simulink model "activeControlSimcopycopy"  (R2026a)
settings: Solver=ode4  StopTime=35  FixedStep=0.01
settings Model: DataDictionary=navParams.sldd  PauseTimes=2  Creator=maxhu  LastModifiedBy=nathanscott

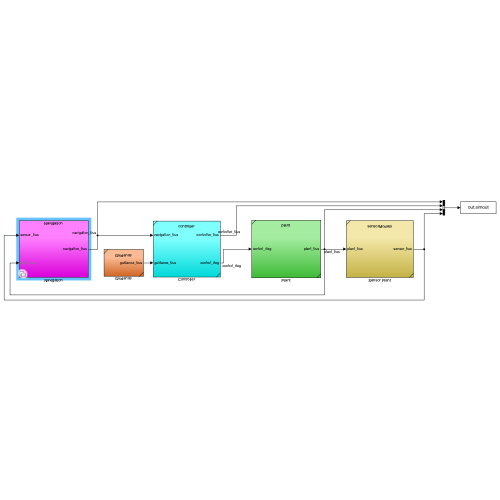
[thumbnail: Simulink's stored preview of the top-level diagram]
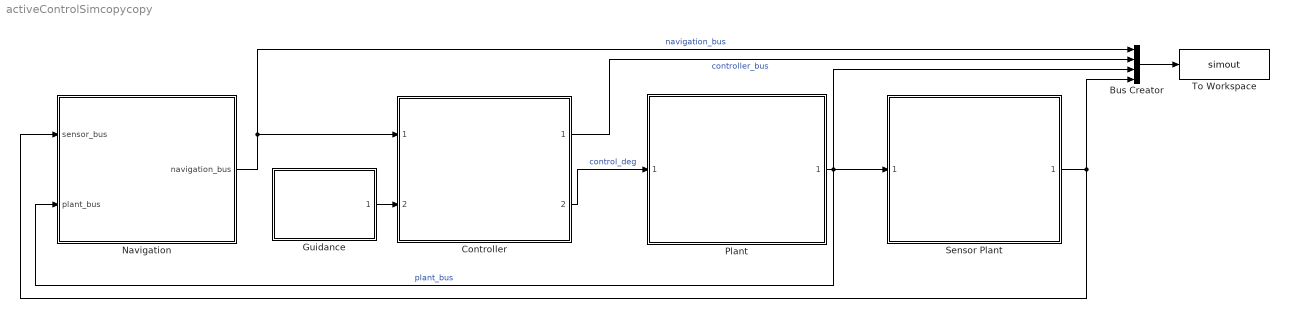
== system activeControlSimcopycopy ==
  Bus Creator : BusCreator  Inputs=4
  Controller : Subsystem  ReferencedSubsystem=controller
      settings: PermitHierarchicalResolution=None
  Guidance : Subsystem  ReferencedSubsystem=Guidance
      settings: PermitHierarchicalResolution=None
  Navigation : Subsystem  Variant=on
  Plant : Subsystem  ReferencedSubsystem=plant
      settings: PermitHierarchicalResolution=None
  Sensor Plant : Subsystem  ReferencedSubsystem=sensorModels
      settings: PermitHierarchicalResolution=None
  To Workspace : ToWorkspace  VariableName=simout  SaveFormat=Timeseries  SampleTime=-1
  wires:
  Plant/1 -> Sensor Plant/1, Bus Creator/3, Navigation/2(plant_bus)  "plant_bus"
  Sensor Plant/1 -> Bus Creator/4, Navigation/1(sensor_bus)
  Bus Creator/1 -> To Workspace/1
  Guidance/1 -> Controller/2
  Navigation/1(navigation_bus) -> Bus Creator/1, Controller/1  "navigation_bus"
  Controller/1 -> Bus Creator/2  "controller_bus"
  Controller/2 -> Plant/1  "control_deg"

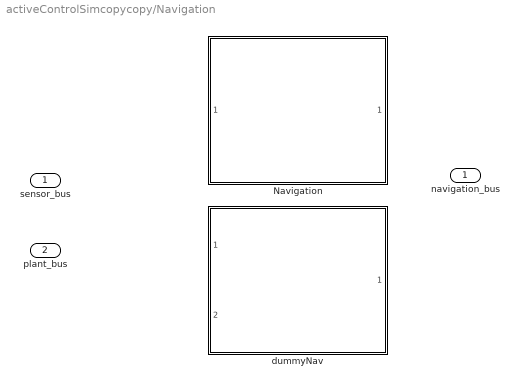
== system activeControlSimcopycopy/Navigation ==
  sensor_bus : Inport
  plant_bus : Inport  Port=2
  Navigation : Subsystem  VariantControl=navControl.useNav_b == true  ReferencedSubsystem=navigation
      settings: PermitHierarchicalResolution=None
  dummyNav : Subsystem  VariantControl=navControl.useNav_b == false  ReferencedSubsystem=dummyNav
  navigation_bus : Outport
